simulink model "simu2"  (R2025b)
settings: Solver=VariableStepAuto  StartTime=0.0  StopTime=10.0  RelTol=1e-3
values from neighbouring files (symbols this model uses):
  g = 9.81    [init_params.m]
  K_lqr = lqr(A, B, Q, R)    [init_params.m]
  m = 0.468    [init_params.m]
settings Model: Creator=ThinkPad  LastModifiedBy=ThinkPad

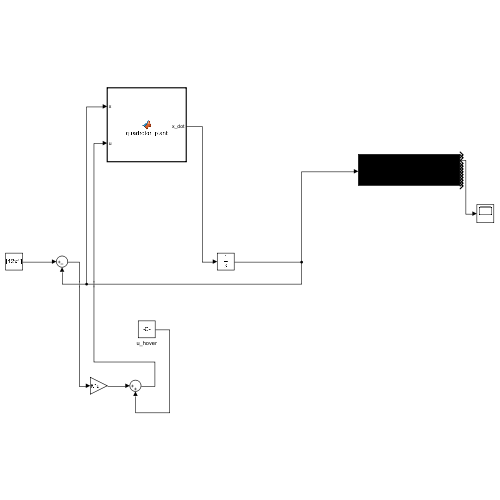
[thumbnail: Simulink's stored preview of the top-level diagram]
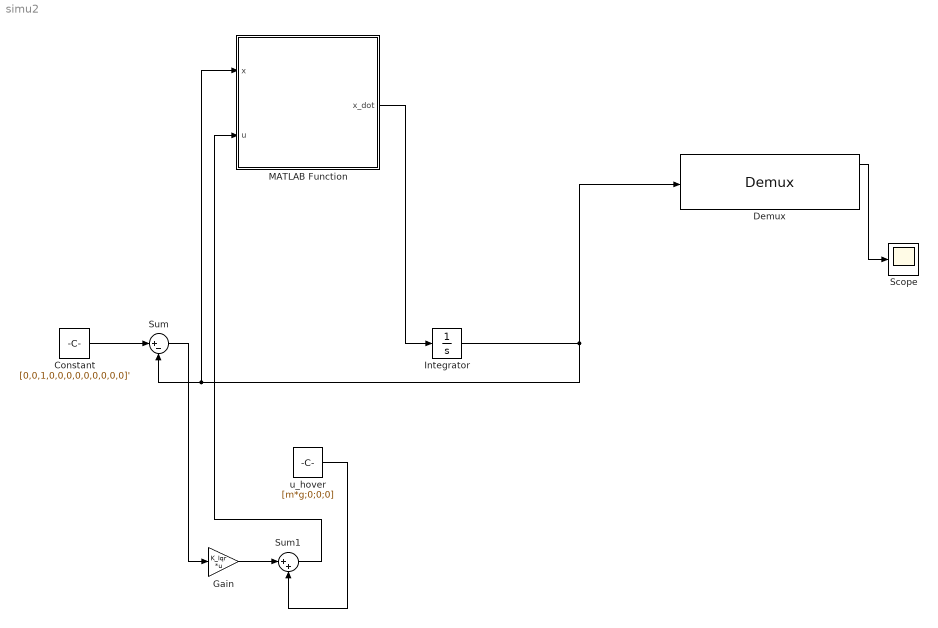
== system simu2 ==
  Constant : Constant  Value=[0,0,1,0,0,0,0,0,0,0,0,0]'
  Demux : Demux  Outputs=12
  Gain : Gain  Gain=K_lqr  Multiplication=Matrix(K*u)
  Integrator : Integrator  InitialCondition=zeros(12,1)
  MATLAB Function : MATLAB Function  TreatAsAtomicUnit=on
  Scope : Scope
      settings: ActiveDisplayYMinimum=-1.6394425357894267  ActiveDisplayYMaximum=3.7142348276888311
  Sum : Sum  Inputs=|+-
  Sum1 : Sum  Inputs=|++
  u_hover : Constant  Value=[m*g;0;0;0]
  wires:
  Sum/1 -> Gain/1
  Gain/1 -> Sum1/1
  u_hover/1 -> Sum1/2
  Constant/1 -> Sum/1
  MATLAB Function/1(x_dot) -> Integrator/1
  Integrator/1 -> MATLAB Function/1(x), Sum/2, Demux/1
  Demux/3 -> Scope/1
  Sum1/1 -> MATLAB Function/2(u)

== matlab function simu2/MATLAB Function ==
  data: x input size=12; u input size=4; x_dot output
function x_dot = quadrotor_plant(x, u)
% 1. Khai báo trực tiếp các thông số vật lý (Tránh tạo cổng thừa)
m  = 0.468;
g  = 9.81;
Ix = 4.856e-3;
Iy = 4.856e-3;
Iz = 8.801e-3;

% 2. Giải nén trạng thái x (Vector 12x1)
phi   = x(4); theta = x(5); psi   = x(6);
dx    = x(7); dy    = x(8); dz    = x(9);
dphi  = x(10); dtheta = x(11); dpsi = x(12);

% 3. Giải nén tín hiệu điều khiển u (Vector 4x1)
ft    = u(1);
tau_x = u(2);
tau_y = u(3);
tau_z = u(4);

% 4. Phương trình gia tốc tịnh tiến & gia tốc góc
ddot_x = -(ft/m) * (sin(phi)*sin(psi) + cos(phi)*cos(psi)*sin(theta));
ddot_y = -(ft/m) * (cos(phi)*sin(psi)*sin(theta) - cos(psi)*sin(phi));
ddot_z = g - (ft/m) * (cos(phi)*cos(theta));

ddot_phi   = ((Iy - Iz)/Ix) * dtheta * dpsi + (1/Ix) * tau_x;
ddot_theta = ((Iz - Ix)/Iy) * dphi * dpsi   + (1/Iy) * tau_y;
ddot_psi   = ((Ix - Iy)/Iz) * dphi * dtheta + (1/Iz) * tau_z;

% 5. Trả về vector x_dot dạng cột (12x1)
x_dot = [dx; dy; dz; dphi; dtheta; dpsi; ddot_x; ddot_y; ddot_z; ddot_phi; ddot_theta; ddot_psi];
end
